simulink model "chaine_qpsk_sim"  (R2023b)
settings: Solver=FixedStepDiscrete  StartTime=0.0  StopTime=Nbq  FixedStep=1  RelTol=1e-3
undefined symbols (not defined in the file): sigq2
settings Model: Creator=e2507457  LastModifiedBy=e2507457

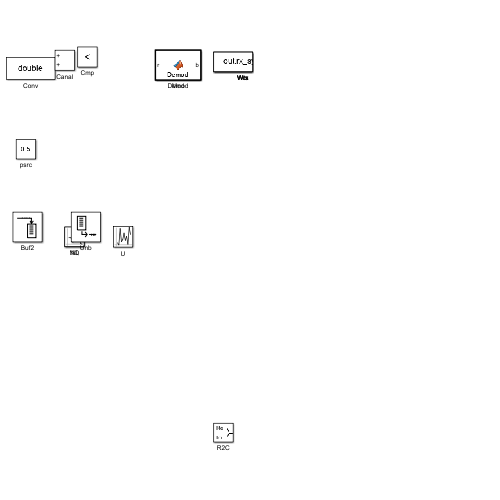
[thumbnail: Simulink's stored preview of the top-level diagram]
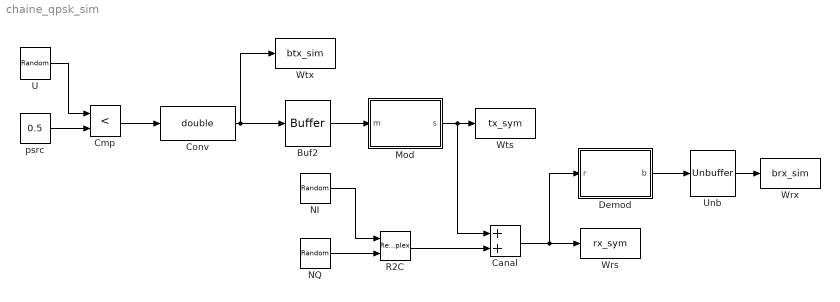
== system chaine_qpsk_sim ==
  Buf2 : Buffer  N=2
  Canal : Sum
  Cmp : RelationalOperator  Operator=<  OutDataTypeStr=boolean  RndMeth=Simplest  InputSameDT=off
  Conv : DataTypeConversion  OutDataTypeStr=double  SaturateOnIntegerOverflow=off  RndMeth=Floor
  Demod : MATLAB Function  TreatAsAtomicUnit=on
  Mod : MATLAB Function  TreatAsAtomicUnit=on
  NI : RandomNumber  Variance=sigq2  Seed=33  SampleTime=2
  NQ : RandomNumber  Variance=sigq2  Seed=34  SampleTime=2
  R2C : RealImagToComplex
  U : UniformRandomNumber  Minimum=0  Seed=32  SampleTime=1
  Unb : Unbuffer
  Wrs : ToWorkspace  VariableName=rx_sym  SampleTime=-1
  Wrx : ToWorkspace  VariableName=brx_sim  SampleTime=-1
  Wts : ToWorkspace  VariableName=tx_sym  SampleTime=-1
  Wtx : ToWorkspace  VariableName=btx_sim  SampleTime=-1
  psrc : Constant  Value=0.5  SampleTime=1
  wires:
  NI/1 -> R2C/1
  NQ/1 -> R2C/2
  U/1 -> Cmp/1
  Conv/1 -> Buf2/1, Wtx/1
  psrc/1 -> Cmp/2
  Buf2/1 -> Mod/1(m)
  Cmp/1 -> Conv/1
  Mod/1(s) -> Canal/1, Wts/1
  R2C/1 -> Canal/2
  Canal/1 -> Demod/1(r), Wrs/1
  Demod/1(b) -> Unb/1
  Unb/1 -> Wrx/1

== matlab function chaine_qpsk_sim/Mod ==
  data: m input; s output
function s = Mod(m)
%#codegen
s = complex((1-2*m(1))/sqrt(2), (1-2*m(2))/sqrt(2));
end

== matlab function chaine_qpsk_sim/Demod ==
  data: r input; b output
function b = Demod(r)
%#codegen
b = [double(real(r) < 0); double(imag(r) < 0)];
end
